simulink model "BESS_GFM_PV_GFL_10kV_Stage1"  (R2026a)
settings: Solver=ode23t  StopTime=0.8  MaxStep=1e-5
InitFcn:
  | run(fullfile(fileparts(get_param(bdroot,'FileName')),'..','scripts','init_bess_pv_stage1.m'));
undefined symbols (not defined in the file): ee_sli_rtmsupport, G, gcbh, S1
libraries: ee_lib x19, nesl_utility x15, fl_lib x14, eeGeneralControl x4, simulink x3, eeTransforms x2, sl_discontinuities x1, sl_signal_attributes x1
(part 2 of 2)

== system BESS_GFM_PV_GFL_10kV_Stage1/03 PV-GFL Branch/Reference_Project_PLL/Subsystem/Sinusoidal Measurement (PLL, Three-Phase)/Input filter/Filter ==
  f : Inport
  u : Inport  Port=2
  Moving Average (Variable Frequency) : eeGeneralControl/Moving Average (Variable Frequency)  VariantControl=Variant1  LabelModeActiveChoice=Discrete  f0=F0  fmin=5  x0=0  BufferSize=8192  Ts=Ts
  Mean : Outport
  wires:
  f/1 -> Moving Average (Variable Frequency)/1
  u/1 -> Moving Average (Variable Frequency)/2
  Moving Average (Variable Frequency)/1 -> Mean/1

== system BESS_GFM_PV_GFL_10kV_Stage1/03 PV-GFL Branch/Reference_Project_PLL/Subsystem/Sinusoidal Measurement (PLL, Three-Phase)/Input filter/Passthrough ==
  f : Inport
  u : Inport  Port=2
  Terminator : Terminator
  Mean : Outport
  wires:
  u/1 -> Mean/1
  f/1 -> Terminator/1

== system BESS_GFM_PV_GFL_10kV_Stage1/03 PV-GFL Branch/Reference_Project_PLL/Subsystem/Sinusoidal Measurement (PLL, Three-Phase)/Normalization/Normalize ==
  q : Inport
  mag : Inport  Port=2
  Mux1 : Mux  Inputs=2
  Normalization : Fcn  Expr=u(2)/(u(1)+(1e-6)*(u(1)==0))
  y : Outport
  wires:
  Normalization/1 -> y/1
  q/1 -> Mux1/2
  mag/1 -> Mux1/1
  Mux1/1 -> Normalization/1

== system BESS_GFM_PV_GFL_10kV_Stage1/03 PV-GFL Branch/Reference_Project_PLL/Subsystem/Sinusoidal Measurement (PLL, Three-Phase)/Normalization/Passthrough ==
  q : Inport
  mag : Inport  Port=2
  Terminator : Terminator
  y : Outport
  wires:
  mag/1 -> Terminator/1
  q/1 -> y/1
